simulink model "emg_project"  (R2026a)
settings: Solver=VariableStepAuto

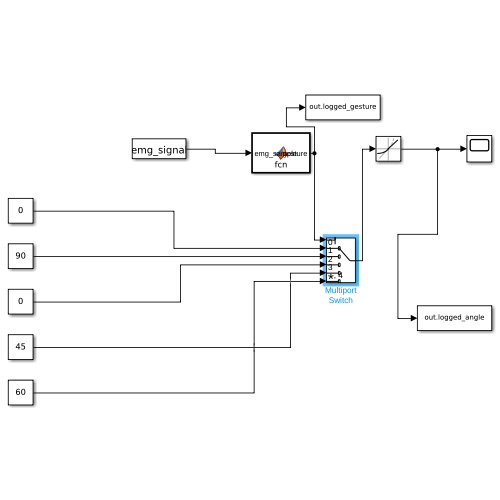
[thumbnail: Simulink's stored preview of the top-level diagram]
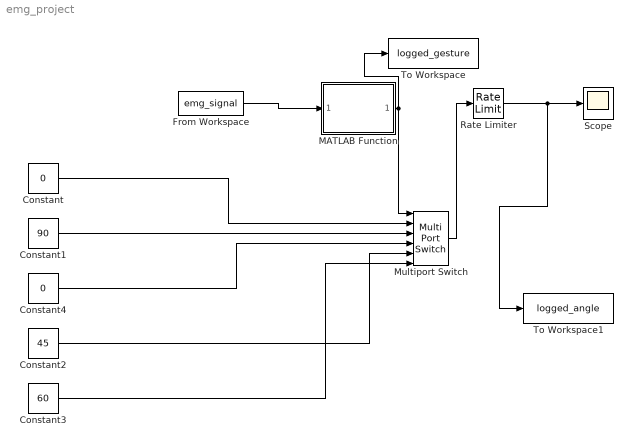
== system emg_project ==
  Constant : Constant  Value=0
  Constant1 : Constant  Value=90
  Constant2 : Constant  Value=45
  Constant3 : Constant  Value=60
  Constant4 : Constant  Value=0
  From Workspace : FromWorkspace  VariableName=emg_signal
  MATLAB Function : MATLAB Function  TreatAsAtomicUnit=on
  Multiport Switch : MultiPortSwitch  DataPortOrder=Zero-based contiguous  Inputs=5  DiagnosticForDefault=None  zeroidx=on  SaturateOnIntegerOverflow=off  InputSameDT=off
  Rate Limiter : RateLimiter  SampleTimeMode=inherited
  Scope : Scope
      settings: ActiveDisplayYMinimum=1.0756065606836454  ActiveDisplayYMaximum=1.1483062387799732
  To Workspace : ToWorkspace  VariableName=logged_gesture  SaveFormat=Timeseries  SampleTime=-1
  To Workspace1 : ToWorkspace  VariableName=logged_angle  SaveFormat=Timeseries  SampleTime=-1
  wires:
  From Workspace/1 -> MATLAB Function/1(emg_sample)
  Rate Limiter/1 -> To Workspace1/1, Scope/1
  MATLAB Function/1(gesture) -> Multiport Switch/1, To Workspace/1
  Constant1/1 -> Multiport Switch/3
  Constant/1 -> Multiport Switch/2
  Constant4/1 -> Multiport Switch/4
  Constant3/1 -> Multiport Switch/6
  Constant2/1 -> Multiport Switch/5
  Multiport Switch/1 -> Rate Limiter/1

== matlab function emg_project/MATLAB Function ==
  data: emg_sample input; gesture output
function gesture = fcn(emg_sample)
coder.extrinsic('predict');
coder.extrinsic('evalin');

gesture = double(0); 

% 1. Reshape the input signal into a row.
x = double(emg_sample(:)'); 

% 2. Calculate features for each channel.
mav     = abs(x);          
rms_val = abs(x);          
wl      = zeros(1, length(x));    
zc      = zeros(1, length(x));    

% 3. Concatenate all features.
combined = [mav, rms_val, wl, zc];
features_all = combined(:)'; 

% 4. Strict check: enforce exactly 40 feature columns.
if length(features_all) ~= 40
    features_40 = zeros(1, 40);
    % Copy available values and pad the remaining entries with zeros.
    len = min(length(features_all), 40);
    features_40(1:len) = features_all(1:len);
else
    features_40 = features_all;
end

pred_gesture = 0; 

% 5. Pass exactly 40 features to the model.
if coder.target('MATLAB') || true
    assignin('base', 'current_features', features_40);
    pred_gesture = evalin('base', 'predict(trainedModel, current_features)');
end

gesture = double(pred_gesture);
end
